simulink model "dc1_op_unlinked_R2016a_alt"  (R2023b)
settings: Solver=FixedStepDiscrete  StartTime=0.0  StopTime=2.5  RelTol=1e-3  EnableMultiTasking=on
InitFcn:
  | Ts_Control=100e-6;
  | Ts_Power=Ts_Control/50;
libraries: spsGroundLib x3, spsParallelRLCBranchLib x2, spsDCVoltageSourceLib x2, spsCurrentMeasurementLib x1, spsDCMachineLib x1, spsOnDelayLib x1, spsStairGeneratorLib x1, spsPWMGeneratorDCDCLib x1, spsTwoQuadrantDCDCConverterLib x1, spsVoltageMeasurementLib x1, sps_lib x1
Description:
  | Copyright 2008-2017 The MathWorks, Inc.
settings Model: Creator=MathWorks  LastModifiedBy=Liu
settings SolverCC: AlgebraicLoopSolver=TrustRegion
settings DataIOCC: LimitDataPoints=on  SaveFormat=Array  SignalLoggingSaveFormat=ModelDataLogs  SaveOutput=off  SignalLogging=off  SaveTime=off  ReturnWorkspaceOutputs=off  SignalLoggingName=sigsOut
settings OptimizationCC: ExpressionDepthLimit=2147483647  InitFltsAndDblsToZero=on  LifeSpan=inf
settings DebuggingCC: UnderspecifiedInitializationDetection=Classic  MergeDetectMultiDrivingBlocksExec=none  CheckExecutionContextPreStartOutputMsg=on  SignalResolutionControl=TryResolveAllWithWarning  MultiTaskDSMMsg=warning  MultiTaskCondExecSysMsg=none  FcnCallInpInsideContextMsg=warning  UnconnectedInputMsg=warning  UnconnectedOutputMsg=warning  UnconnectedLineMsg=warning  StateNameClashWarn=warning  SFUnexpectedBacktrackingDiag=warning  SFNoUnconditionalDefaultTransitionDiag=warning  ArithmeticOperatorsInVariantConditions=warning
settings HardwareCC: ProdBitPerPointer=32  ProdBitPerSizeT=32  ProdBitPerPtrDiffT=32  ProdLargestAtomicFloat=None  ProdIntDivRoundTo=Undefined  ProdEndianess=Unspecified  ProdWordSize=32  ProdHWDeviceType=32-bit Generic  TargetUnknown=on
settings ModelReferenceCC: EnableRefExpFcnMdlSchedulingChecks=on  PropagateSignalLabelsOutOfModel=off
settings SFSimCC: SimUseLocalCustomCode=off  CustomCodeUndefinedFunction=UseInterfaceOnly
settings RTWCC: RTWUseLocalCustomCode=off
settings CodeAppCC: StateflowObjectComments=on
settings GRTTargetCC: TargetLangStandard=C89/C90 (ANSI)  CombineOutputUpdateFcns=off  GRTInterface=on
settings ConfigComp: CovMetricSettings=dw  CovSaveCumulativeToWorkspaceVar=on  CovSaveSingleToWorkspaceVar=on  CovExternalEMLEnable=off  CovSFcnEnable=off
settings SimscapeCC: SimscapeNormalizeSystem=off

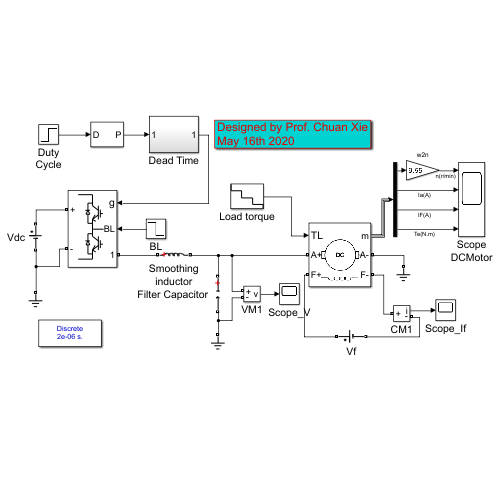
[thumbnail: Simulink's stored preview of the top-level diagram]
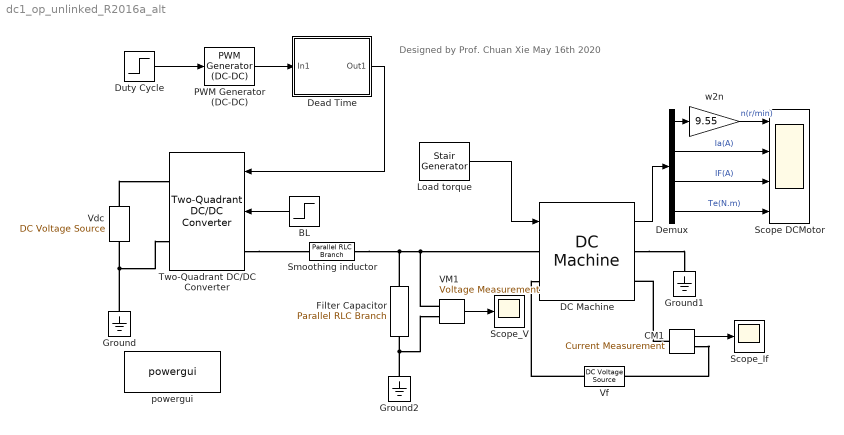
== system dc1_op_unlinked_R2016a_alt ==
  note: Designed by Prof. Chuan Xie
      | May 16th 2020
  BL : Step  Time=0.2  Before=1  After=0  SampleTime=Ts_Power
  CM1 : spsCurrentMeasurementLib/Current Measurement  PhasorSimulation=off  OutputType=Complex  PSBequivalent=0
  DC Machine : spsDCMachineLib/DC Machine  PresetModel=02: 5HP 240V 1750RPM Field:150V  MechanicalLoad=Torque TL  FieldType=Wound  ShowDetailedParameters=on  MeasurementBus=off  RLa=[0.78 0.016]  RLf=[150 112.5]  Laf=1.234  MachineConstant=Torque constant (N.m/A)  Ke=1.8  Kt=1.8  J=0.05  Bm=0.01  Tf=0  w0=1800/9.55  Ifinit=0.8  TsPowergui=0  TsBlock=-1
  Dead Time : Subsystem
  Demux : Demux
  Duty Cycle : Step  Time=0.01  After=0.6  SampleTime=Ts_Power
  Filter Capacitor : spsParallelRLCBranchLib/Parallel RLC Branch  LConnTagsString=a  RConnTagsString=__new0  BranchType=C  Resistance=[]  Inductance=0.5e-3  SetiL0=off  InitialCurrent=0  Capacitance=100e-6  Setx0=off  InitialVoltage=0  Measurements=None
  Ground : spsGroundLib/Ground  LConnTagsString=a
  Ground1 : spsGroundLib/Ground  LConnTagsString=a
  Ground2 : spsGroundLib/Ground  LConnTagsString=a
  Load torque : spsStairGeneratorLib/Stair Generator  t=[0, 0.5, 1, 1.5 2]  e=[1, 0.75, 0.5, 0.25, 0.1]*20.46  Ts=0
  PWM Generator (DC-DC) : spsPWMGeneratorDCDCLib/PWM Generator (DC-DC)  Fsw=10e3  Ts=Ts_Power
  Scope DCMotor : Scope  NumInputPorts=4
  Scope_If : Scope
  Scope_V : Scope
  Smoothing inductor : spsParallelRLCBranchLib/Parallel RLC Branch  LConnTagsString=a  RConnTagsString=__new0  BranchType=L  Resistance=[]  Inductance=5e-3  SetiL0=off  InitialCurrent=0  Capacitance=[]  Setx0=off  InitialVoltage=0  Measurements=None
  Two-Quadrant DC/DC Converter : spsTwoQuadrantDCDCConverterLib/Two-Quadrant DC//DC Converter  ModelType=Switching devices  Ron=0.5  Rs=1e6  Cs=inf  Vforward=[0,0]  Ron_Diode=1e-3  Rs_Diode=1e6  Cs_Diode=inf  Vf_Diode=1e-3  Rs_CurrentSource=inf  Ron_ACsource=1e-3
      settings: LibrarySourceBlock=|
      | sps_lib/Power Electronics/Two-Quadrant
      | DC//DC Converter
  VM1 : spsVoltageMeasurementLib/Voltage Measurement  PhasorSimulation=off  OutputType=Complex  PSBequivalent=0
  Vdc : spsDCVoltageSourceLib/DC Voltage Source  Description=source block  Amplitude=300  Measurements=None
      settings: AttributesFormatString=\n
  Vf : spsDCVoltageSourceLib/DC Voltage Source  Description=source block  Amplitude=120  Measurements=None
      settings: AttributesFormatString=\n
  powergui : sps_lib/powergui  Priority=2  SimulationMode=Discrete  SampleTime=Ts_Power  frequency=60  Iterations=50  frequencyindice=0  Pbase=100e6  ErrMax=1e-4  UnitsV=kV  UnitsW=MW  buscounter=0  FunctionMessages=off  echomessages=off  EnableUseOfTLC=off  CurrentSourceSwitches=off  DisableSnubberDevices=off  DisableRonSwitches=off  DisableVfSwitches=off  DisplayEquations=off  AutomaticDiscreteSolvers=off  SolverType=Tustin/Backward Euler (TBE)  Interpol=off  ExternalGateDelay=off  methode=off  Ts=0  x0status=blocks  SPID=off  SwTol=0  HookPort=off  NonlinearTolerance=1e-4  nMaxIteration=100  ContinueOnMaxIteration=off  RestoreLinks=warning  ResistiveCurrentMeasurement=off  Frange=[0:2:500]  Ylog=off  Xlog=on  ShowGrid=off  save=off  variable=ZData  structure=0  ZoomFFT=on  StartTime=0.0  cycles=1  DisplayStyle=1  fundamental=60  FreqAxis=off  MaxFrequency=1000  frequencyindicesteady=1  RmsSteady=1  display=off
  w2n : Gain  Gain=9.55
  wires:
  Demux/1 -> w2n/1
  Demux/2 -> Scope DCMotor/2  "Ia(A)"
  Demux/3 -> Scope DCMotor/3  "IF(A)"
  Demux/4 -> Scope DCMotor/4  "Te(N.m)"
  w2n/1 -> Scope DCMotor/1  "n(r/min)"
  VM1/1 -> Scope_V/1
  Duty Cycle/1 -> PWM Generator (DC-DC)/1
  PWM Generator (DC-DC)/1 -> Dead Time/1(In1)
  Dead Time/1(Out1) -> Two-Quadrant DC/DC Converter/1
  BL/1 -> Two-Quadrant DC/DC Converter/2
  Load torque/1 -> DC Machine/1
  DC Machine/1 -> Demux/1
  CM1/1 -> Scope_If/1
  connections:
  Vdc/RConn1 -- Two-Quadrant DC/DC Converter/RConn1
  Ground/LConn1 -- Two-Quadrant DC/DC Converter/RConn2 -- Vdc/LConn1
  DC Machine/RConn1 -- Ground1/LConn1
  Two-Quadrant DC/DC Converter/LConn1 -- Smoothing inductor/LConn1
  Smoothing inductor/RConn1 -- VM1/LConn1 -- DC Machine/LConn1 -- Filter Capacitor/LConn1
  Ground2/LConn1 -- VM1/LConn2 -- Filter Capacitor/RConn1
  Vf/RConn1 -- DC Machine/LConn2
  CM1/RConn1 -- Vf/LConn1
  CM1/LConn1 -- DC Machine/RConn2

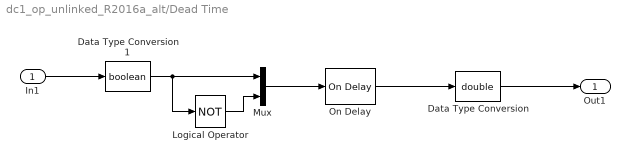
== system dc1_op_unlinked_R2016a_alt/Dead Time ==
  In1 : Inport
  Data Type Conversion : DataTypeConversion  OutDataTypeStr=double  SaturateOnIntegerOverflow=off  RndMeth=Floor
  Data Type Conversion1 : DataTypeConversion  OutDataTypeStr=boolean  SaturateOnIntegerOverflow=off  RndMeth=Floor
  Logical Operator : Logic  Operator=NOT  AllPortsSameDT=off  OutDataTypeStr=boolean
  Mux : Mux  Inputs=2
  On Delay : spsOnDelayLib/On Delay  DelayType=On delay  delay=Ts_Power*2  ic=0  Ts=Ts_Power
  Out1 : Outport
  wires:
  In1/1 -> Data Type Conversion1/1
  Logical Operator/1 -> Mux/2
  On Delay/1 -> Data Type Conversion/1
  Mux/1 -> On Delay/1
  Data Type Conversion1/1 -> Logical Operator/1, Mux/1
  Data Type Conversion/1 -> Out1/1
